simulink model "voo"  (R2026a)
settings: Solver=VariableStepAuto  StopTime=100
values from neighbouring files (symbols this model uses):
  g = 9.8    [rocket.m]
  Mf = 50    [rocket.m]
  SRef = pi*DRef^2/4    (= 0.011689866264)    [rocket.m]
  TabProp = [   0            F     MProp0 ;      Tqf          F     0;            Tqf + 0.01   0     0]    [rocket.m]
  VCd = [  0    0.33;      0.7  0.33;      0.9  0.42;      1.1  0.67;      1.2  0.68;      1.5  0.7]    [rocket.m]
libraries: aerolibptmass x2, aerolibatmos2 x1, simulink x1

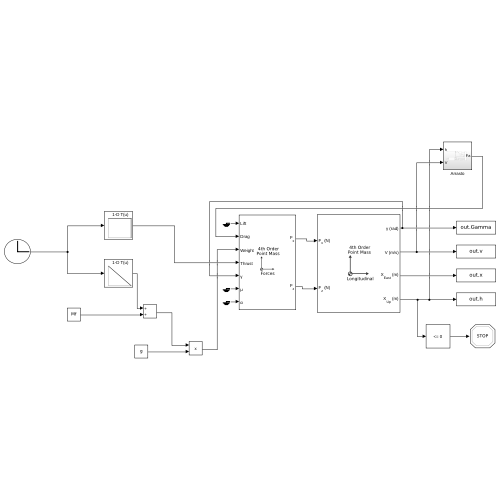
[thumbnail: Simulink's stored preview of the top-level diagram]
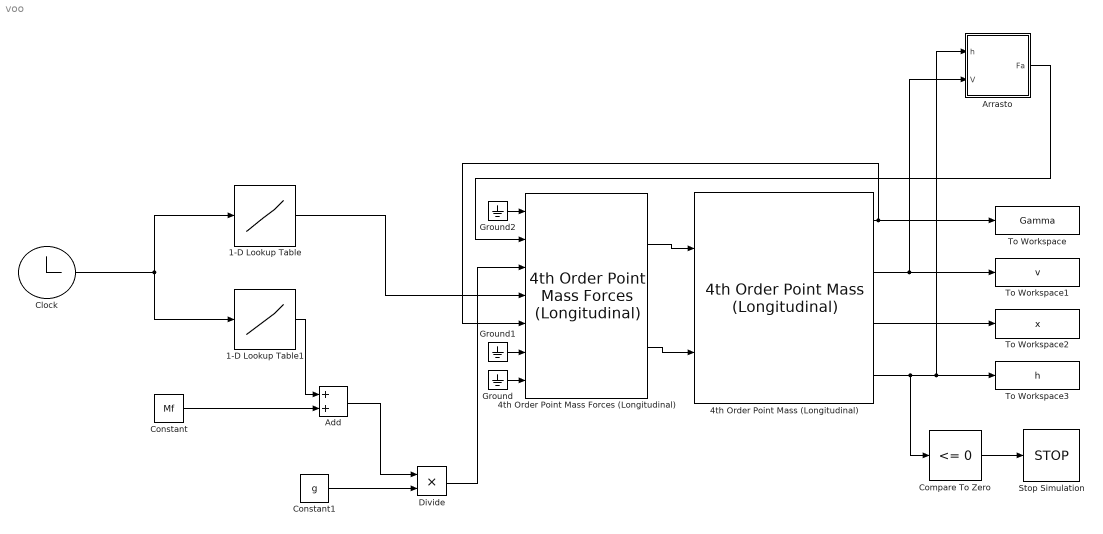
== system voo ==
  1-D Lookup Table : Lookup_n-D  NumberOfTableDimensions=1  BreakpointsForDimension1=TabProp(:,1)  Table=TabProp(:,2)  ExtrapMethod=Clip  InternalRulePriority=Speed  RndMeth=Simplest
  1-D Lookup Table1 : Lookup_n-D  NumberOfTableDimensions=1  BreakpointsForDimension1=TabProp(:,1)  Table=TabProp(:,3)  ExtrapMethod=Clip  InternalRulePriority=Speed  RndMeth=Simplest
  4th Order Point Mass (Longitudinal) : aerolibptmass/4th Order Point Mass (Longitudinal)  units=Metric (MKS)  gamma0=Gamma0  V0=V0  x0=x0  h0=h0  mass0=M0
  4th Order Point Mass Forces (Longitudinal) : aerolibptmass/4th Order Point Mass Forces (Longitudinal)
  Add : Sum
  Arrasto : Subsystem
  Clock : Clock
  Compare To Zero : simulink/Logic and Bit Operations/Compare To Zero  relop=<=  OutDataTypeStr=boolean
  Constant : Constant  Value=Mf
  Constant1 : Constant  Value=g
  Divide : Product  Inputs=**
  Ground : Ground
  Ground1 : Ground
  Ground2 : Ground
  Stop Simulation : Stop
  To Workspace : ToWorkspace  VariableName=Gamma  SaveFormat=Timeseries  SampleTime=-1
  To Workspace1 : ToWorkspace  VariableName=v  SaveFormat=Timeseries  SampleTime=-1
  To Workspace2 : ToWorkspace  VariableName=x  SaveFormat=Timeseries  SampleTime=-1
  To Workspace3 : ToWorkspace  VariableName=h  SaveFormat=Timeseries  SampleTime=-1
  wires:
  4th Order Point Mass Forces (Longitudinal)/2 -> 4th Order Point Mass (Longitudinal)/2
  4th Order Point Mass Forces (Longitudinal)/1 -> 4th Order Point Mass (Longitudinal)/1
  Add/1 -> Divide/1
  Constant/1 -> Add/2
  Constant1/1 -> Divide/2
  1-D Lookup Table1/1 -> Add/1
  1-D Lookup Table/1 -> 4th Order Point Mass Forces (Longitudinal)/4
  Divide/1 -> 4th Order Point Mass Forces (Longitudinal)/3
  4th Order Point Mass (Longitudinal)/1 -> To Workspace/1, 4th Order Point Mass Forces (Longitudinal)/5
  Ground2/1 -> 4th Order Point Mass Forces (Longitudinal)/1
  Ground1/1 -> 4th Order Point Mass Forces (Longitudinal)/6
  Ground/1 -> 4th Order Point Mass Forces (Longitudinal)/7
  Clock/1 -> 1-D Lookup Table1/1, 1-D Lookup Table/1
  4th Order Point Mass (Longitudinal)/4 -> Compare To Zero/1, To Workspace3/1, Arrasto/1(h)
  4th Order Point Mass (Longitudinal)/2 -> To Workspace1/1, Arrasto/2(V)
  Arrasto/1(Fa) -> 4th Order Point Mass Forces (Longitudinal)/2
  4th Order Point Mass (Longitudinal)/3 -> To Workspace2/1
  Compare To Zero/1 -> Stop Simulation/1

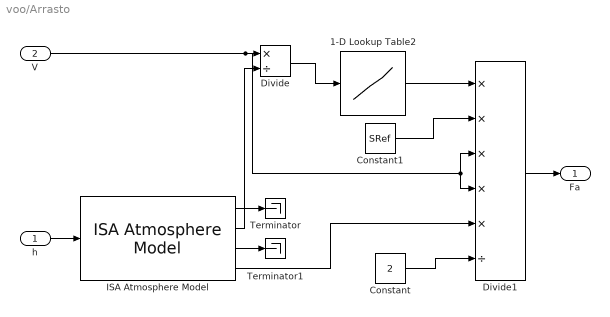
== system voo/Arrasto ==
  h : Inport
  V : Inport  Port=2
  1-D Lookup Table2 : Lookup_n-D  NumberOfTableDimensions=1  BreakpointsForDimension1=VCd(:,1)  Table=VCd(:,2)  ExtrapMethod=Clip  InternalRulePriority=Speed  RndMeth=Simplest
  Constant : Constant  Value=2
  Constant1 : Constant  Value=SRef
  Divide : Product  Inputs=*/
  Divide1 : Product  Inputs=*****/
  ISA Atmosphere Model : aerolibatmos2/ISA Atmosphere Model  useExtended=off  action=None  custom=off  viscosityOut=off  g=9.80665  gamma=1.4  R=287.0531  L=0.0065  h_trop=11000  h_strat=20000  rho0=1.225  P0=101325  T0=288.15  h0=0  S=110.4  Tref=273.15  muref=1.716e-5
  Terminator : Terminator
  Terminator1 : Terminator
  Fa : Outport
  wires:
  h/1 -> ISA Atmosphere Model/1
  ISA Atmosphere Model/1 -> Terminator/1
  ISA Atmosphere Model/3 -> Terminator1/1
  V/1 -> Divide1/3, Divide1/4, Divide/1
  ISA Atmosphere Model/2 -> Divide/2
  Constant/1 -> Divide1/6
  ISA Atmosphere Model/4 -> Divide1/5
  Divide/1 -> 1-D Lookup Table2/1
  1-D Lookup Table2/1 -> Divide1/1
  Constant1/1 -> Divide1/2
  Divide1/1 -> Fa/1
